simulink model "TSPMe_power"  (R2023a)
settings: Solver=VariableStepAuto  StartTime=0.0  StopTime=16000  RelTol=1e-3
libraries: fl_lib x8, nesl_utility x7, BatteryLibrary_lib x2
settings Model: Creator=widana_d  LastModifiedBy=widana_d
settings DebuggingCC: UnconnectedInputMsg=warning  UnconnectedOutputMsg=warning  UnconnectedLineMsg=warning
settings ModelReferenceCC: EnableRefExpFcnMdlSchedulingChecks=on
settings RTWCC: DLArmComputeVersion=19.05

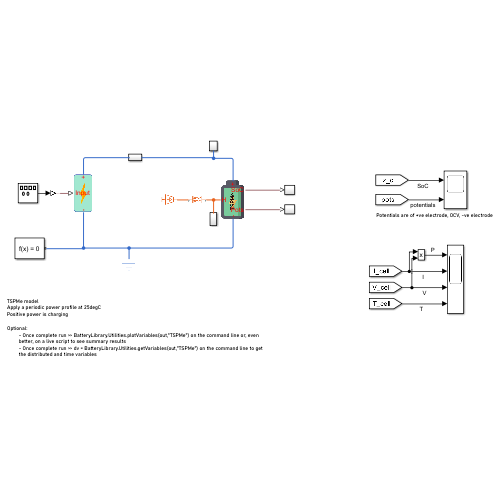
[thumbnail: Simulink's stored preview of the top-level diagram]
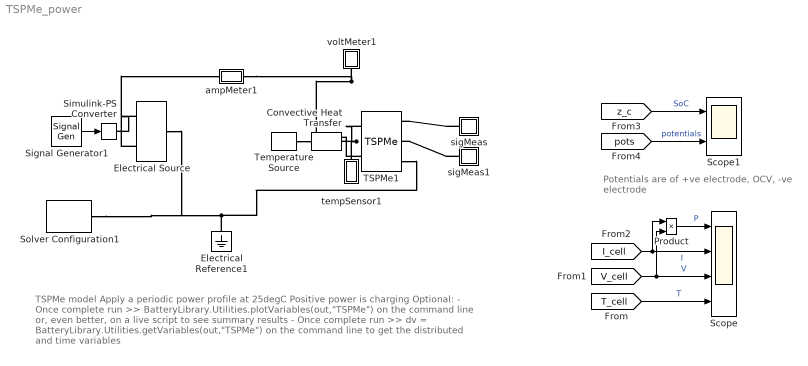
== system TSPMe_power ==
  note: TSPMe model
      | Apply a periodic power profile at 25degC
      | Positive power is charging
      |
      | Optional:
      | - Once complete run >> BatteryLibrary.Utilities.plotVariables(out,"TSPMe") on the command line or, even better, on a live script to see summary results
      | - Once complete run >> dv = BatteryLibrary.Utilities.getVariables(out,"TSPMe") on the command line to get the distributed and time variables
  note: Potentials are of +ve electrode, OCV, -ve electrode
  Convective Heat Transfer : fl_lib/Thermal/Thermal Elements/Convective Heat Transfer  thermal_type=foundation.enum.constant_variable.constant  area=0.0046 m^2  heat_tr_coeff=35 W/(m^2 * K)  min_heat_tr_coeff=1e-3 W/(K*m^2)  T_specify=off  T_priority=None  T=0 K  T_nominal_specify=off  T_nominal_unit=K  T_nominal_value=1  Q_specify=off  Q_priority=None  Q=0 W  Q_nominal_specify=off  Q_nominal_unit=W  Q_nominal_value=1
  Electrical Reference1 : fl_lib/Electrical/Electrical Elements/Electrical Reference
  Electrical Source : BatteryLibrary_lib/Utilities/Electrical Source  inType=2
      settings: InternalSimscapePortConfiguration="{\"Bottom\":[{\"id\":\"n\",\"label\":\"-\",\"type\":\"foundation.electrical.electrical\"}],\"Left\":[{\"id\":\"inputSignal\",\"label\":\"Input\",\"type\":\"input\"}],\"Right\":[],\"Top\":[{\"id\":\"p\",\"label\":\"+\",\"type\":\"foundation.electrical.electrical\"}]}"
  Product : Product
  Scope : Scope  NumInputPorts=4
  Scope1 : Scope  NumInputPorts=2
  Signal Generator1 : SignalGenerator  WaveForm=square  Amplitude=8  Frequency=62E-6
  Simulink-PS Converter : nesl_utility/Simulink-PS Converter  PhysicalDomain=network_engine_domain  SubClassName=ps_input  LeftPortType=input  RightPortType=output  PseudoPeriodic=off  Frequencies=[]  NoiseDistribution=none  NoiseParameters=[]  Unit=1  AffineConversion=off  FilteringAndDerivatives=provide  SimscapeFilterOrder=1  InputFilterTimeConstant=0.001  UdotUserProvided=0
  Solver Configuration1 : nesl_utility/Solver Configuration  PhysicalDomain=network_engine_domain  SubClassName=solver  LeftPortType=input  RightPortType=generic  Tones=[]  Harmonics=[]  SimulateNoise=off  Profile=off  UseLocalSampling=off  EnableSwitchedLinearOptims=on  FrequencyDomain=off  UseCCode=off  RelTol=0.001  AbsTol=1e-06  MinStep=1e-09  ToWorkspace=off  RevertToSquareIcSolve=off  NumHomotopyIterations=100  PhasorMode=off  PhasorModeNumHarmonics=1  ConsistencySolver=NEWTON_FTOL  IndexReductionMethod=DerivativeReplacement  DoDC=off  ResidualTolerance=1e-09  ConsistencyTolSource=GLOBAL  ConsistencyAbsTol=0.001  ConsistencyRelTol=0.001  ConsistencyTolFactor=0.001  UseLocalSolver=off  LocalSolverChoice=NE_BACKWARD_EULER_ADVANCER  ResolveIndetEquations=on  FunctionEvalNumThread=1  LocalSolverSampleTime=0.001  DoFixedCost=off  MaxNonlinIter=3  MaxModeIter=2  ComputeImpulses=off  ImpulseIterations=2  LinearAlgebra=auto  LinearAlgebraNumThread=0  EquationFormulation=NE_TIME_EF  DelaysMemoryBudget=1024  AutomaticFiltering=on  FilteringTimeConstant=0.001  PartitionStorageMethod=AS_NEEDED  PartitionMemoryBudget=1024  PartitionMethod=ROBUST
  TSPMe1 : BatteryLibrary_lib/Models/TSPMe  z0=1  T0=25 degC  Cn=4.9 hr*A  DnRef=3.3E-14 m^2/s  DpRef=4E-15 m^2/s  sigma_nRef=215 S/m  sigma_eRef=1.2 S/m  sigma_pRef=0.18 S/m  tr=0.2594  ce0=1000 mol/m^3  cn_max=33133 mol/m^3  cp_max=63104 mol/m^3  sn_max=0.9014  sn_min=0.0279  sp_max=0.9072  sp_min=0.2567  knRef=6.48E-7 m^2.50000*A/mol^1.50000  kpRef=3.42E-6 m^2.50000*A/mol^1.50000  Cp=110 J/K  Tref=298 K  Ea_kn=1 kJ/mol  Ea_kp=1 kJ/mol  Ea_Dn=75 kJ/mol  Ea_Dp=10 kJ/mol  Ea_De=1.2 kJ/mol  Ea_sigman=80 kJ/mol  Ea_sigmae=80 kJ/mol  Ea_sigmap=80 kJ/mol  Ln=85.2 um  Ls=12 um  Lp=75.6 um  Area_p=1027 cm^2  eps_n=0.25  eps_s=0.47  eps_p=0.335  Rn=5.86 um  Rp=5.22 um  an=3.84E5 1/m  ap=3.82E5 1/m
      settings: InternalSimscapePortConfiguration="{\"Bottom\":[{\"id\":\"n\",\"label\":\"-\",\"type\":\"foundation.electrical.electrical\"}],\"Left\":[{\"id\":\"Hi\",\"label\":\"H\",\"type\":\"foundation.thermal.thermal\"}],\"Right\":[{\"id\":\"z\",\"label\":\"SoC\",\"type\":\"output\"},{\"id\":\"pots\",\"label\":\"Pots\",\"type\":\"output\"}],\"Top\":[{\"id\":\"p\",\"label\":\"+\",\"type\":\"foundation.electrical.electrical\"}]}"
  Temperature Source : fl_lib/Thermal/Thermal Sources/Temperature Source  temperature=25 degC
  ampMeter1 : Subsystem
  sigMeas : Subsystem
  sigMeas1 : Subsystem
  tempSensor1 : Subsystem
  voltMeter1 : Subsystem
  wires:
  [z_c] -> Scope1/1  "SoC"
  [pots] -> Scope1/2  "potentials"
  [T_cell] -> Scope/4  "T"
  [I_cell] -> Product/1, Scope/2  "I"
  [V_cell] -> Product/2, Scope/3  "V"
  Product/1 -> Scope/1  "P"
  Signal Generator1/1 -> Simulink-PS Converter/1
  connections:
  Convective Heat Transfer/LConn1 -- TSPMe1/LConn1 -- tempSensor1/LConn1
  Electrical Reference1/LConn1 -- TSPMe1/RConn3 -- Electrical Source/RConn1 -- Solver Configuration1/RConn1
  voltMeter1/LConn1 -- TSPMe1/LConn2 -- ampMeter1/RConn1
  Temperature Source/LConn1 -- Convective Heat Transfer/RConn1
  Electrical Source/LConn2 -- ampMeter1/LConn1
  sigMeas/LConn1 -- TSPMe1/RConn1
  sigMeas1/LConn1 -- TSPMe1/RConn2
  Electrical Source/LConn1 -- Simulink-PS Converter/RConn1

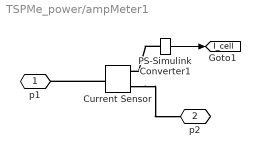
== system TSPMe_power/ampMeter1 ==
  Current Sensor : fl_lib/Electrical/Electrical Sensors/Current Sensor
  PS-Simulink Converter1 : nesl_utility/PS-Simulink Converter  PhysicalDomain=network_engine_domain  SubClassName=ps_output  LeftPortType=input  RightPortType=output  PseudoPeriodic=off  Frequencies=[]  VectorFormat=1-D array  Unit=inherit  AffineConversion=off
  p1 : PMIOPort  Side=Left
  p2 : PMIOPort  Port=2  Side=Right
  tag scope: I_cell=global
  wires:
  PS-Simulink Converter1/1 -> [I_cell]
  connections:
  Current Sensor/RConn2 -- p2/RConn1
  Current Sensor/LConn1 -- p1/RConn1
  PS-Simulink Converter1/LConn1 -- Current Sensor/RConn1

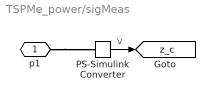
== system TSPMe_power/sigMeas ==
  PS-Simulink Converter : nesl_utility/PS-Simulink Converter  PhysicalDomain=network_engine_domain  SubClassName=ps_output  LeftPortType=input  RightPortType=output  PseudoPeriodic=off  Frequencies=[]  VectorFormat=1-D array  Unit=inherit  AffineConversion=off
  p1 : PMIOPort  Side=Left
  tag scope: z_c=global
  wires:
  PS-Simulink Converter/1 -> [z_c]  "V"
  connections:
  p1/RConn1 -- PS-Simulink Converter/LConn1

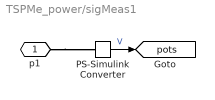
== system TSPMe_power/sigMeas1 ==
  PS-Simulink Converter : nesl_utility/PS-Simulink Converter  PhysicalDomain=network_engine_domain  SubClassName=ps_output  LeftPortType=input  RightPortType=output  PseudoPeriodic=off  Frequencies=[]  VectorFormat=1-D array  Unit=inherit  AffineConversion=off
  p1 : PMIOPort  Side=Left
  tag scope: pots=global
  wires:
  PS-Simulink Converter/1 -> [pots]  "V"
  connections:
  p1/RConn1 -- PS-Simulink Converter/LConn1

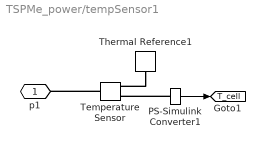
== system TSPMe_power/tempSensor1 ==
  PS-Simulink Converter1 : nesl_utility/PS-Simulink Converter  PhysicalDomain=network_engine_domain  SubClassName=ps_output  LeftPortType=input  RightPortType=output  PseudoPeriodic=off  Frequencies=[]  VectorFormat=1-D array  Unit=inherit  AffineConversion=off
  Temperature Sensor : fl_lib/Thermal/Thermal Sensors/Temperature Sensor  temperature_measure=foundation.enum.MeasurementReference.difference
  Thermal Reference1 : fl_lib/Thermal/Thermal Elements/Thermal Reference
  p1 : PMIOPort  Side=Left
  tag scope: T_cell=global
  wires:
  PS-Simulink Converter1/1 -> [T_cell]
  connections:
  Temperature Sensor/LConn1 -- p1/RConn1
  PS-Simulink Converter1/LConn1 -- Temperature Sensor/RConn2
  Thermal Reference1/LConn1 -- Temperature Sensor/RConn1

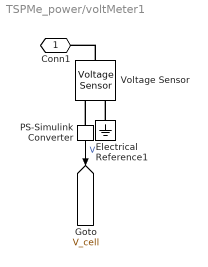
== system TSPMe_power/voltMeter1 ==
  Electrical Reference1 : fl_lib/Electrical/Electrical Elements/Electrical Reference
  PS-Simulink Converter : nesl_utility/PS-Simulink Converter  PhysicalDomain=network_engine_domain  SubClassName=ps_output  LeftPortType=input  RightPortType=output  PseudoPeriodic=off  Frequencies=[]  VectorFormat=1-D array  Unit=inherit  AffineConversion=off
  Voltage Sensor : fl_lib/Electrical/Electrical Sensors/Voltage Sensor
  Conn1 : PMIOPort  Side=Left
  tag scope: V_cell=global
  wires:
  PS-Simulink Converter/1 -> [V_cell]  "V"
  connections:
  Voltage Sensor/LConn1 -- Conn1/RConn1
  PS-Simulink Converter/LConn1 -- Voltage Sensor/RConn1
  Electrical Reference1/LConn1 -- Voltage Sensor/RConn2
